simulink model "DATA_PERTURB_AND_OBSERVE_STEADY_STATE_IRRADIATION_VARIATION"  (R2023b)
settings: Solver=ode23  StartTime=0.0  StopTime=0.5  RelTol=1e-7
undefined symbols (not defined in the file): Acid, Lead
libraries: spsMeanLib x40, spsSeriesRLCBranchLib x25, spsVoltageMeasurementLib x20, spsCurrentMeasurementLib x10, spsBatteryLib x5, spsDiodeLib x5, spsMosfetLib x5, simulink x5, spsPVArrayLib x5, spsPWMGeneratorDCDCLib x5, sps_lib x1
settings Model: Creator=User  LastModifiedBy=D E L L
settings DebuggingCC: AlgebraicLoopMsg=none

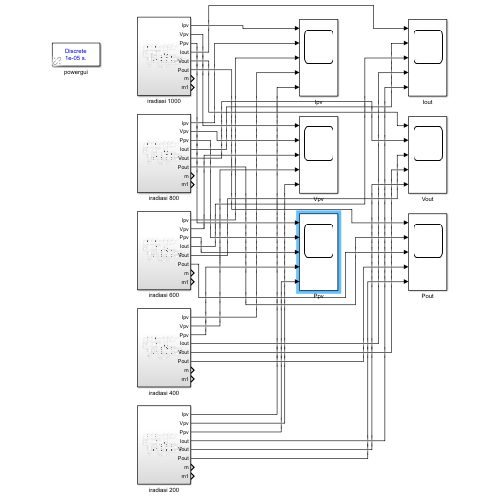
[thumbnail: Simulink's stored preview of the top-level diagram]
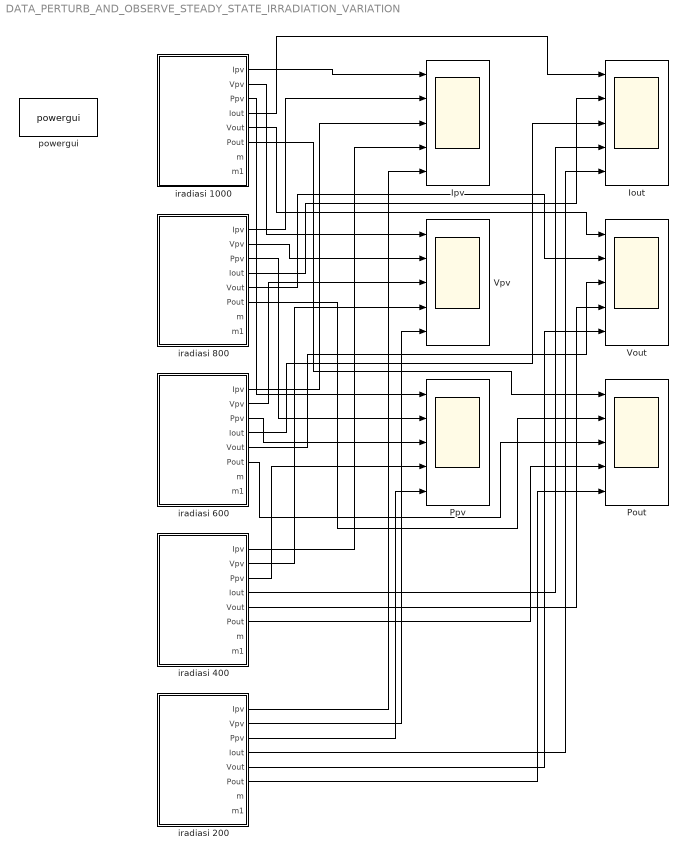
== system DATA_PERTURB_AND_OBSERVE_STEADY_STATE_IRRADIATION_VARIATION ==
  Iout : Scope  NumInputPorts=5
  Ipv : Scope  NumInputPorts=5
  Pout : Scope  NumInputPorts=5
  Ppv : Scope  NumInputPorts=5
  Vout : Scope  NumInputPorts=5
  Vpv : Scope  NumInputPorts=5
  iradiasi 1000 : Subsystem
  iradiasi 200 : Subsystem
  iradiasi 400 : Subsystem
  iradiasi 600 : Subsystem
  iradiasi 800 : Subsystem
  powergui : sps_lib/powergui  Priority=1  SimulationMode=Discrete  SampleTime=1e-05  frequency=60  Iterations=50  frequencyindice=0  Pbase=100e6  ErrMax=1e-4  UnitsV=kV  UnitsW=MW  buscounter=0  FunctionMessages=off  echomessages=off  EnableUseOfTLC=off  CurrentSourceSwitches=off  DisableSnubberDevices=off  DisableRonSwitches=off  DisableVfSwitches=off  DisplayEquations=off  AutomaticDiscreteSolvers=off  SolverType=Tustin/Backward Euler (TBE)  Interpol=off  ExternalGateDelay=off  methode=off  Ts=100  x0status=blocks  SPID=on  SwTol=0  HookPort=off  NonlinearTolerance=1e-4  nMaxIteration=100  ContinueOnMaxIteration=off  RestoreLinks=warning  ResistiveCurrentMeasurement=off  Frange=[0:2:500]  Ylog=off  Xlog=on  ShowGrid=off  save=off  variable=ZData  structure=0  ZoomFFT=off  StartTime=0.0  cycles=1  DisplayStyle=1  fundamental=60  FreqAxis=off  MaxFrequency=1000  frequencyindicesteady=1  RmsSteady=1  display=off
  wires:
  iradiasi 1000/1(Ipv) -> Ipv/1
  iradiasi 800/1(Ipv) -> Ipv/2
  iradiasi 600/1(Ipv) -> Ipv/3
  iradiasi 400/1(Ipv) -> Ipv/4
  iradiasi 200/1(Ipv) -> Ipv/5
  iradiasi 1000/2(Vpv) -> Vpv/1
  iradiasi 800/2(Vpv) -> Vpv/2
  iradiasi 600/2(Vpv) -> Vpv/3
  iradiasi 400/2(Vpv) -> Vpv/4
  iradiasi 200/2(Vpv) -> Vpv/5
  iradiasi 1000/3(Ppv) -> Ppv/1
  iradiasi 800/3(Ppv) -> Ppv/2
  iradiasi 600/3(Ppv) -> Ppv/3
  iradiasi 400/3(Ppv) -> Ppv/4
  iradiasi 200/3(Ppv) -> Ppv/5
  iradiasi 1000/4(Iout) -> Iout/1
  iradiasi 800/4(Iout) -> Iout/2
  iradiasi 600/4(Iout) -> Iout/3
  iradiasi 400/4(Iout) -> Iout/4
  iradiasi 200/4(Iout) -> Iout/5
  iradiasi 1000/5(Vout) -> Vout/1
  iradiasi 800/5(Vout) -> Vout/2
  iradiasi 600/5(Vout) -> Vout/3
  iradiasi 400/5(Vout) -> Vout/4
  iradiasi 200/5(Vout) -> Vout/5
  iradiasi 1000/6(Pout) -> Pout/1
  iradiasi 800/6(Pout) -> Pout/2
  iradiasi 600/6(Pout) -> Pout/3
  iradiasi 400/6(Pout) -> Pout/4
  iradiasi 200/6(Pout) -> Pout/5

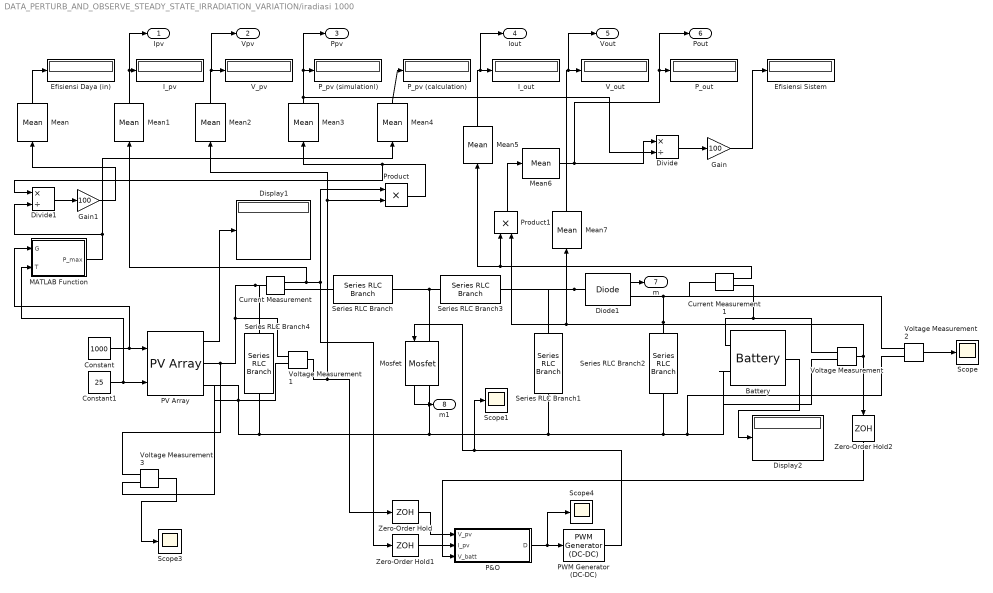
== system DATA_PERTURB_AND_OBSERVE_STEADY_STATE_IRRADIATION_VARIATION/iradiasi 1000 ==
  Battery : spsBatteryLib/Battery  BatType=Lead-Acid  ShowTempParam=off  ThermalPreset=no  ShowAgeParam=off  NomV=12  NomQ=3.5  SOC=90  Batt_Tr=1  PresetModel=off  MaxQ=3.125  MinV=9  FullV=14.4  Dis_rate=0.6  R=0.04  Normal_OP=0.93083  expZone="[12.2171         0.01]"  current=[6.5 13 32.5]  Units=Time  Tci=20  NomT=20  T2=-30  MaxQ2=4.8  FullV2=7.1  Normal_OP2=5.655  expZone2="[6.58           1]"  Rca=0.6  ti=2000  Dp=0  Neq0=0  Tsim=1e6  Ta1=25  Qeol=5.4*0.9  Reol=0.013333*1.2  Char_age=[2.3478, 3]  Dis_age=[2.3478, 10]  N1=1500  N2=10500  N3=1000  N4=1400  Ta2=45  N5=950
  Constant : Constant  Value=1000
  Constant1 : Constant  Value=25
  Current Measurement : spsCurrentMeasurementLib/Current Measurement  PhasorSimulation=off  OutputType=Complex  PSBequivalent=0
  Current Measurement1 : spsCurrentMeasurementLib/Current Measurement  PhasorSimulation=off  OutputType=Complex  PSBequivalent=0
  Diode1 : spsDiodeLib/Diode  Ron=0.001  Lon=0  Vf=0.4  IC=0  UseSnubber=0  Rs=500  Cs=250e-9  Measurements=on
  Display1 : Display
  Display2 : Display
  Divide : Product  Inputs=*/
  Divide1 : Product  Inputs=*/
  Efisiensi Daya (in) : Display
  Efisiensi Sistem : Display
  Gain : Gain  Gain=100
  Gain1 : Gain  Gain=100
  I_out : Display
  I_pv : Display
  MATLAB Function : MATLAB Function  TreatAsAtomicUnit=on
  Mean{,1..7} (8 alike) : spsMeanLib/Mean  Freq=60  Vinit=0  Ts=0
  Mosfet : spsMosfetLib/Mosfet  Ron=0.044  Lon=0  Rd=1.3  Vfd=0  IC=0  Rs=1e5  Cs=inf  Measurements=on
  P&O : Subsystem
  PV Array : spsPVArrayLib/PV Array  Npar=1  Nser=1  PlotType=array @ 1000 W/m2 & specified temperatures  S_vec="[ 1000  500  100 ]"  Temp_C_vec="[ 45 25  ]"  ModuleName=User-defined  PlotWhenSelected=off  Pm=10.08  Ncell=36  Voc=21.6  Isc=0.61  Vm=18  Im=0.56  beta_Voc_pc=-0.36099  alpha_Isc_pc=0.102  beta_Voc=-0.077974  alpha_Isc=0.0006222  IL=0.61115  I0=2.2544e-11  nI=0.97389  Rsh=828.4328  Rs=1.5603  RobustModel=off  RobustCellTemperature=313.3991  BAL=on  Tc=1e-6  Tfilter=1e-5
  PWM Generator (DC-DC) : spsPWMGeneratorDCDCLib/PWM Generator (DC-DC)  Fsw=31000  Ts=0
  P_out : Display
  P_pv (calculation) : Display
  P_pv (simulationl) : Display
  Product : Product
  Product1 : Product
  Scope{,1,3..4} (4 alike) : Scope
  Series RLC Branch : spsSeriesRLCBranchLib/Series RLC Branch  LConnTagsString=__new0  RConnTagsString=__new0  BranchType=L  Resistance=1  Inductance=1.5e-3  SetiL0=on  InitialCurrent=0.01  Capacitance=1e-6  Setx0=off  InitialVoltage=0  Measurements=None
  Series RLC Branch1 : spsSeriesRLCBranchLib/Series RLC Branch  LConnTagsString=__new0  RConnTagsString=__new0  BranchType=L  Resistance=1  Inductance=1.5e-3  SetiL0=on  InitialCurrent=0.01  Capacitance=1e-6  Setx0=off  InitialVoltage=0  Measurements=None
  Series RLC Branch2 : spsSeriesRLCBranchLib/Series RLC Branch  LConnTagsString=__new0  RConnTagsString=__new0  BranchType=C  Resistance=1  Inductance=1e-3  SetiL0=off  InitialCurrent=0  Capacitance=470e-6  Setx0=on  InitialVoltage=0.1  Measurements=None
  Series RLC Branch3 : spsSeriesRLCBranchLib/Series RLC Branch  LConnTagsString=__new0  RConnTagsString=__new0  BranchType=C  Resistance=1  Inductance=1e-3  SetiL0=off  InitialCurrent=0  Capacitance=22e-6  Setx0=off  InitialVoltage=0  Measurements=None
  Series RLC Branch4 : spsSeriesRLCBranchLib/Series RLC Branch  LConnTagsString=__new0  RConnTagsString=__new0  BranchType=C  Resistance=1  Inductance=1e-3  SetiL0=off  InitialCurrent=0  Capacitance=470e-6  Setx0=on  InitialVoltage=0.1  Measurements=None
  V_out : Display
  V_pv : Display
  Voltage Measurement{,1..3} (4 alike) : spsVoltageMeasurementLib/Voltage Measurement  PhasorSimulation=off  OutputType=Complex  PSBequivalent=0
  Zero-Order Hold : ZeroOrderHold  SampleTime=0.05
  Zero-Order Hold1 : ZeroOrderHold  SampleTime=0.05
  Zero-Order Hold2 : ZeroOrderHold  SampleTime=0.05
  Ipv : Outport
  Vpv : Outport  Port=2
  Ppv : Outport  Port=3
  Iout : Outport  Port=4
  Vout : Outport  Port=5
  Pout : Outport  Port=6
  m : Outport  Port=7
  m1 : Outport  Port=8
  wires:
  Mean1/1 -> Ipv/1, I_pv/1
  Mean2/1 -> Vpv/1, V_pv/1
  PWM Generator (DC-DC)/1 -> Scope1/1, Mosfet/1
  Divide/1 -> Gain/1
  Current Measurement1/1 -> Product1/1, Mean5/1
  Constant1/1 -> MATLAB Function/2(T), PV Array/2
  Constant/1 -> MATLAB Function/1(G), PV Array/1
  Divide1/1 -> Gain1/1
  Gain1/1 -> Mean/1
  Voltage Measurement2/1 -> Scope/1
  Voltage Measurement/1 -> Product1/2, Mean7/1, Zero-Order Hold2/1
  Diode1/1 -> m/1
  Gain/1 -> Efisiensi Sistem/1
  P&O/1(D) -> Scope4/1, PWM Generator (DC-DC)/1
  Product/1 -> Mean3/1, Divide1/1
  Voltage Measurement1/1 -> Zero-Order Hold/1, Mean2/1, Product/2
  Current Measurement/1 -> Zero-Order Hold1/1, Product/1, Mean1/1
  Mean6/1 -> Divide/1, Pout/1, P_out/1
  Mean4/1 -> P_pv (calculation)/1
  Zero-Order Hold2/1 -> P&O/3(V_batt)
  Product1/1 -> Mean6/1
  Zero-Order Hold1/1 -> P&O/2(I_pv)
  Mean3/1 -> Ppv/1, P_pv (simulationl)/1, Divide/2
  Zero-Order Hold/1 -> P&O/1(V_pv)
  Mean5/1 -> Iout/1, I_out/1
  Voltage Measurement3/1 -> Scope3/1
  Mean7/1 -> Vout/1, V_out/1
  MATLAB Function/1(P_max) -> Mean4/1, Divide1/2
  Battery/1 -> Display2/1
  PV Array/1 -> Display1/1
  Mean/1 -> Efisiensi Daya (in)/1
  Mosfet/1 -> m1/1
  connections:
  Diode1/LConn1 -- Series RLC Branch3/RConn1 -- Series RLC Branch1/LConn1
  Series RLC Branch1/RConn1 -- Series RLC Branch4/RConn1 -- Voltage Measurement3/LConn2 -- PV Array/RConn2 -- Voltage Measurement1/LConn2 -- Mosfet/RConn1 -- Voltage Measurement2/LConn2 -- Voltage Measurement/LConn2 -- Battery/LConn2 -- Series RLC Branch2/RConn1
  PV Array/RConn1 -- Voltage Measurement3/LConn1 -- Voltage Measurement1/LConn1 -- Series RLC Branch4/LConn1 -- Current Measurement/LConn1
  Series RLC Branch3/LConn1 -- Series RLC Branch/RConn1 -- Mosfet/LConn1
  Series RLC Branch2/LConn1 -- Current Measurement1/LConn1 -- Voltage Measurement2/LConn1 -- Diode1/RConn1
  Current Measurement/RConn1 -- Series RLC Branch/LConn1
  Current Measurement1/RConn1 -- Voltage Measurement/LConn1 -- Battery/LConn1

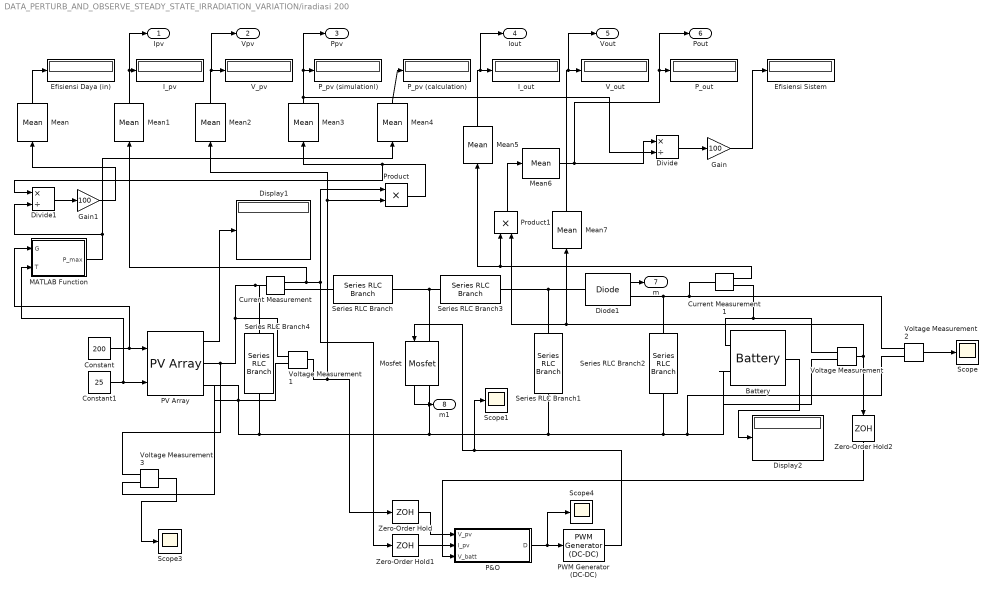
== system DATA_PERTURB_AND_OBSERVE_STEADY_STATE_IRRADIATION_VARIATION/iradiasi 200 ==
  Battery : spsBatteryLib/Battery  BatType=Lead-Acid  ShowTempParam=off  ThermalPreset=no  ShowAgeParam=off  NomV=12  NomQ=3.5  SOC=90  Batt_Tr=1  PresetModel=off  MaxQ=3.125  MinV=9  FullV=14.4  Dis_rate=0.6  R=0.04  Normal_OP=0.93083  expZone="[12.2171         0.01]"  current=[6.5 13 32.5]  Units=Time  Tci=20  NomT=20  T2=-30  MaxQ2=4.8  FullV2=7.1  Normal_OP2=5.655  expZone2="[6.58           1]"  Rca=0.6  ti=2000  Dp=0  Neq0=0  Tsim=1e6  Ta1=25  Qeol=5.4*0.9  Reol=0.013333*1.2  Char_age=[2.3478, 3]  Dis_age=[2.3478, 10]  N1=1500  N2=10500  N3=1000  N4=1400  Ta2=45  N5=950
  Constant : Constant  Value=200
  Constant1 : Constant  Value=25
  Current Measurement : spsCurrentMeasurementLib/Current Measurement  PhasorSimulation=off  OutputType=Complex  PSBequivalent=0
  Current Measurement1 : spsCurrentMeasurementLib/Current Measurement  PhasorSimulation=off  OutputType=Complex  PSBequivalent=0
  Diode1 : spsDiodeLib/Diode  Ron=0.001  Lon=0  Vf=0.4  IC=0  UseSnubber=0  Rs=500  Cs=250e-9  Measurements=on
  Display1 : Display
  Display2 : Display
  Divide : Product  Inputs=*/
  Divide1 : Product  Inputs=*/
  Efisiensi Daya (in) : Display
  Efisiensi Sistem : Display
  Gain : Gain  Gain=100
  Gain1 : Gain  Gain=100
  I_out : Display
  I_pv : Display
  MATLAB Function : MATLAB Function  TreatAsAtomicUnit=on
  Mean{,1..7} (8 alike) : spsMeanLib/Mean  Freq=60  Vinit=0  Ts=0
  Mosfet : spsMosfetLib/Mosfet  Ron=0.044  Lon=0  Rd=1.3  Vfd=0  IC=0  Rs=1e5  Cs=inf  Measurements=on
  P&O : Subsystem
  PV Array : spsPVArrayLib/PV Array  Npar=1  Nser=1  PlotType=array @ 1000 W/m2 & specified temperatures  S_vec="[ 1000  500  100 ]"  Temp_C_vec="[ 45 25  ]"  ModuleName=User-defined  PlotWhenSelected=off  Pm=10.08  Ncell=36  Voc=21.6  Isc=0.61  Vm=18  Im=0.56  beta_Voc_pc=-0.36099  alpha_Isc_pc=0.102  beta_Voc=-0.077974  alpha_Isc=0.0006222  IL=0.61115  I0=2.2544e-11  nI=0.97389  Rsh=828.4328  Rs=1.5603  RobustModel=off  RobustCellTemperature=313.3991  BAL=on  Tc=1e-6  Tfilter=1e-5
  PWM Generator (DC-DC) : spsPWMGeneratorDCDCLib/PWM Generator (DC-DC)  Fsw=31000  Ts=0
  P_out : Display
  P_pv (calculation) : Display
  P_pv (simulationl) : Display
  Product : Product
  Product1 : Product
  Scope{,1,3..4} (4 alike) : Scope
  Series RLC Branch : spsSeriesRLCBranchLib/Series RLC Branch  LConnTagsString=__new0  RConnTagsString=__new0  BranchType=L  Resistance=1  Inductance=1.5e-3  SetiL0=on  InitialCurrent=0.01  Capacitance=1e-6  Setx0=off  InitialVoltage=0  Measurements=None
  Series RLC Branch1 : spsSeriesRLCBranchLib/Series RLC Branch  LConnTagsString=__new0  RConnTagsString=__new0  BranchType=L  Resistance=1  Inductance=1.5e-3  SetiL0=on  InitialCurrent=0.01  Capacitance=1e-6  Setx0=off  InitialVoltage=0  Measurements=None
  Series RLC Branch2 : spsSeriesRLCBranchLib/Series RLC Branch  LConnTagsString=__new0  RConnTagsString=__new0  BranchType=C  Resistance=1  Inductance=1e-3  SetiL0=off  InitialCurrent=0  Capacitance=470e-6  Setx0=on  InitialVoltage=0.1  Measurements=None
  Series RLC Branch3 : spsSeriesRLCBranchLib/Series RLC Branch  LConnTagsString=__new0  RConnTagsString=__new0  BranchType=C  Resistance=1  Inductance=1e-3  SetiL0=off  InitialCurrent=0  Capacitance=22e-6  Setx0=off  InitialVoltage=0  Measurements=None
  Series RLC Branch4 : spsSeriesRLCBranchLib/Series RLC Branch  LConnTagsString=__new0  RConnTagsString=__new0  BranchType=C  Resistance=1  Inductance=1e-3  SetiL0=off  InitialCurrent=0  Capacitance=470e-6  Setx0=on  InitialVoltage=0.1  Measurements=None
  V_out : Display
  V_pv : Display
  Voltage Measurement{,1..3} (4 alike) : spsVoltageMeasurementLib/Voltage Measurement  PhasorSimulation=off  OutputType=Complex  PSBequivalent=0
  Zero-Order Hold : ZeroOrderHold  SampleTime=0.05
  Zero-Order Hold1 : ZeroOrderHold  SampleTime=0.05
  Zero-Order Hold2 : ZeroOrderHold  SampleTime=0.05
  Ipv : Outport
  Vpv : Outport  Port=2
  Ppv : Outport  Port=3
  Iout : Outport  Port=4
  Vout : Outport  Port=5
  Pout : Outport  Port=6
  m : Outport  Port=7
  m1 : Outport  Port=8
  wires:
  Mean1/1 -> Ipv/1, I_pv/1
  Mean2/1 -> Vpv/1, V_pv/1
  PWM Generator (DC-DC)/1 -> Scope1/1, Mosfet/1
  Divide/1 -> Gain/1
  Current Measurement1/1 -> Product1/1, Mean5/1
  Constant1/1 -> MATLAB Function/2(T), PV Array/2
  Constant/1 -> MATLAB Function/1(G), PV Array/1
  Divide1/1 -> Gain1/1
  Gain1/1 -> Mean/1
  Voltage Measurement2/1 -> Scope/1
  Voltage Measurement/1 -> Product1/2, Mean7/1, Zero-Order Hold2/1
  Diode1/1 -> m/1
  Gain/1 -> Efisiensi Sistem/1
  P&O/1(D) -> Scope4/1, PWM Generator (DC-DC)/1
  Product/1 -> Mean3/1, Divide1/1
  Voltage Measurement1/1 -> Zero-Order Hold/1, Mean2/1, Product/2
  Current Measurement/1 -> Zero-Order Hold1/1, Product/1, Mean1/1
  Mean6/1 -> Divide/1, Pout/1, P_out/1
  Mean4/1 -> P_pv (calculation)/1
  Zero-Order Hold2/1 -> P&O/3(V_batt)
  Product1/1 -> Mean6/1
  Zero-Order Hold1/1 -> P&O/2(I_pv)
  Mean3/1 -> Ppv/1, P_pv (simulationl)/1, Divide/2
  Zero-Order Hold/1 -> P&O/1(V_pv)
  Mean5/1 -> Iout/1, I_out/1
  Voltage Measurement3/1 -> Scope3/1
  Mean7/1 -> Vout/1, V_out/1
  MATLAB Function/1(P_max) -> Mean4/1, Divide1/2
  Battery/1 -> Display2/1
  PV Array/1 -> Display1/1
  Mean/1 -> Efisiensi Daya (in)/1
  Mosfet/1 -> m1/1
  connections:
  Series RLC Branch3/RConn1 -- Diode1/LConn1 -- Series RLC Branch1/LConn1
  Series RLC Branch1/RConn1 -- Series RLC Branch4/RConn1 -- Voltage Measurement3/LConn2 -- PV Array/RConn2 -- Voltage Measurement1/LConn2 -- Mosfet/RConn1 -- Voltage Measurement2/LConn2 -- Voltage Measurement/LConn2 -- Battery/LConn2 -- Series RLC Branch2/RConn1
  PV Array/RConn1 -- Voltage Measurement3/LConn1 -- Voltage Measurement1/LConn1 -- Series RLC Branch4/LConn1 -- Current Measurement/LConn1
  Series RLC Branch/RConn1 -- Series RLC Branch3/LConn1 -- Mosfet/LConn1
  Current Measurement1/LConn1 -- Voltage Measurement2/LConn1 -- Series RLC Branch2/LConn1 -- Diode1/RConn1
  Current Measurement/RConn1 -- Series RLC Branch/LConn1
  Current Measurement1/RConn1 -- Voltage Measurement/LConn1 -- Battery/LConn1

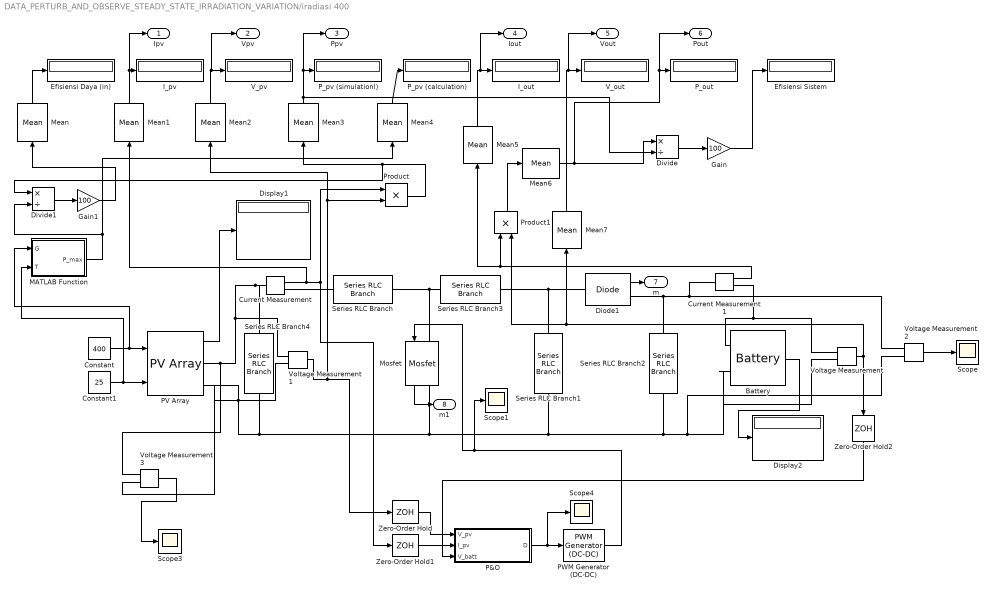
== system DATA_PERTURB_AND_OBSERVE_STEADY_STATE_IRRADIATION_VARIATION/iradiasi 400 ==
  Battery : spsBatteryLib/Battery  BatType=Lead-Acid  ShowTempParam=off  ThermalPreset=no  ShowAgeParam=off  NomV=12  NomQ=3.5  SOC=90  Batt_Tr=1  PresetModel=off  MaxQ=3.125  MinV=9  FullV=14.4  Dis_rate=0.6  R=0.04  Normal_OP=0.93083  expZone="[12.2171         0.01]"  current=[6.5 13 32.5]  Units=Time  Tci=20  NomT=20  T2=-30  MaxQ2=4.8  FullV2=7.1  Normal_OP2=5.655  expZone2="[6.58           1]"  Rca=0.6  ti=2000  Dp=0  Neq0=0  Tsim=1e6  Ta1=25  Qeol=5.4*0.9  Reol=0.013333*1.2  Char_age=[2.3478, 3]  Dis_age=[2.3478, 10]  N1=1500  N2=10500  N3=1000  N4=1400  Ta2=45  N5=950
  Constant : Constant  Value=400
  Constant1 : Constant  Value=25
  Current Measurement : spsCurrentMeasurementLib/Current Measurement  PhasorSimulation=off  OutputType=Complex  PSBequivalent=0
  Current Measurement1 : spsCurrentMeasurementLib/Current Measurement  PhasorSimulation=off  OutputType=Complex  PSBequivalent=0
  Diode1 : spsDiodeLib/Diode  Ron=0.001  Lon=0  Vf=0.4  IC=0  UseSnubber=0  Rs=500  Cs=250e-9  Measurements=on
  Display1 : Display
  Display2 : Display
  Divide : Product  Inputs=*/
  Divide1 : Product  Inputs=*/
  Efisiensi Daya (in) : Display
  Efisiensi Sistem : Display
  Gain : Gain  Gain=100
  Gain1 : Gain  Gain=100
  I_out : Display
  I_pv : Display
  MATLAB Function : MATLAB Function  TreatAsAtomicUnit=on
  Mean{,1..7} (8 alike) : spsMeanLib/Mean  Freq=60  Vinit=0  Ts=0
  Mosfet : spsMosfetLib/Mosfet  Ron=0.044  Lon=0  Rd=1.3  Vfd=0  IC=0  Rs=1e5  Cs=inf  Measurements=on
  P&O : Subsystem
  PV Array : spsPVArrayLib/PV Array  Npar=1  Nser=1  PlotType=array @ 1000 W/m2 & specified temperatures  S_vec="[ 1000  500  100 ]"  Temp_C_vec="[ 45 25  ]"  ModuleName=User-defined  PlotWhenSelected=off  Pm=10.08  Ncell=36  Voc=21.6  Isc=0.61  Vm=18  Im=0.56  beta_Voc_pc=-0.36099  alpha_Isc_pc=0.102  beta_Voc=-0.077974  alpha_Isc=0.0006222  IL=0.61115  I0=2.2544e-11  nI=0.97389  Rsh=828.4328  Rs=1.5603  RobustModel=off  RobustCellTemperature=313.3991  BAL=on  Tc=1e-6  Tfilter=1e-5
  PWM Generator (DC-DC) : spsPWMGeneratorDCDCLib/PWM Generator (DC-DC)  Fsw=31000  Ts=0
  P_out : Display
  P_pv (calculation) : Display
  P_pv (simulationl) : Display
  Product : Product
  Product1 : Product
  Scope{,1,3..4} (4 alike) : Scope
  Series RLC Branch : spsSeriesRLCBranchLib/Series RLC Branch  LConnTagsString=__new0  RConnTagsString=__new0  BranchType=L  Resistance=1  Inductance=1.5e-3  SetiL0=on  InitialCurrent=0.01  Capacitance=1e-6  Setx0=off  InitialVoltage=0  Measurements=None
  Series RLC Branch1 : spsSeriesRLCBranchLib/Series RLC Branch  LConnTagsString=__new0  RConnTagsString=__new0  BranchType=L  Resistance=1  Inductance=1.5e-3  SetiL0=on  InitialCurrent=0.01  Capacitance=1e-6  Setx0=off  InitialVoltage=0  Measurements=None
  Series RLC Branch2 : spsSeriesRLCBranchLib/Series RLC Branch  LConnTagsString=__new0  RConnTagsString=__new0  BranchType=C  Resistance=1  Inductance=1e-3  SetiL0=off  InitialCurrent=0  Capacitance=470e-6  Setx0=on  InitialVoltage=0.1  Measurements=None
  Series RLC Branch3 : spsSeriesRLCBranchLib/Series RLC Branch  LConnTagsString=__new0  RConnTagsString=__new0  BranchType=C  Resistance=1  Inductance=1e-3  SetiL0=off  InitialCurrent=0  Capacitance=22e-6  Setx0=off  InitialVoltage=0  Measurements=None
  Series RLC Branch4 : spsSeriesRLCBranchLib/Series RLC Branch  LConnTagsString=__new0  RConnTagsString=__new0  BranchType=C  Resistance=1  Inductance=1e-3  SetiL0=off  InitialCurrent=0  Capacitance=470e-6  Setx0=on  InitialVoltage=0.1  Measurements=None
  V_out : Display
  V_pv : Display
  Voltage Measurement{,1..3} (4 alike) : spsVoltageMeasurementLib/Voltage Measurement  PhasorSimulation=off  OutputType=Complex  PSBequivalent=0
  Zero-Order Hold : ZeroOrderHold  SampleTime=0.05
  Zero-Order Hold1 : ZeroOrderHold  SampleTime=0.05
  Zero-Order Hold2 : ZeroOrderHold  SampleTime=0.05
  Ipv : Outport
  Vpv : Outport  Port=2
  Ppv : Outport  Port=3
  Iout : Outport  Port=4
  Vout : Outport  Port=5
  Pout : Outport  Port=6
  m : Outport  Port=7
  m1 : Outport  Port=8
  wires:
  Mean1/1 -> Ipv/1, I_pv/1
  Mean2/1 -> Vpv/1, V_pv/1
  PWM Generator (DC-DC)/1 -> Scope1/1, Mosfet/1
  Divide/1 -> Gain/1
  Current Measurement1/1 -> Product1/1, Mean5/1
  Constant1/1 -> MATLAB Function/2(T), PV Array/2
  Constant/1 -> MATLAB Function/1(G), PV Array/1
  Divide1/1 -> Gain1/1
  Gain1/1 -> Mean/1
  Voltage Measurement2/1 -> Scope/1
  Voltage Measurement/1 -> Product1/2, Mean7/1, Zero-Order Hold2/1
  Diode1/1 -> m/1
  Gain/1 -> Efisiensi Sistem/1
  P&O/1(D) -> Scope4/1, PWM Generator (DC-DC)/1
  Product/1 -> Mean3/1, Divide1/1
  Voltage Measurement1/1 -> Zero-Order Hold/1, Mean2/1, Product/2
  Current Measurement/1 -> Zero-Order Hold1/1, Product/1, Mean1/1
  Mean6/1 -> Divide/1, Pout/1, P_out/1
  Mean4/1 -> P_pv (calculation)/1
  Zero-Order Hold2/1 -> P&O/3(V_batt)
  Product1/1 -> Mean6/1
  Zero-Order Hold1/1 -> P&O/2(I_pv)
  Mean3/1 -> Ppv/1, P_pv (simulationl)/1, Divide/2
  Zero-Order Hold/1 -> P&O/1(V_pv)
  Mean5/1 -> Iout/1, I_out/1
  Voltage Measurement3/1 -> Scope3/1
  Mean7/1 -> Vout/1, V_out/1
  MATLAB Function/1(P_max) -> Mean4/1, Divide1/2
  Battery/1 -> Display2/1
  PV Array/1 -> Display1/1
  Mean/1 -> Efisiensi Daya (in)/1
  Mosfet/1 -> m1/1
  connections:
  Series RLC Branch3/RConn1 -- Diode1/LConn1 -- Series RLC Branch1/LConn1
  Series RLC Branch1/RConn1 -- Series RLC Branch4/RConn1 -- Voltage Measurement3/LConn2 -- PV Array/RConn2 -- Voltage Measurement1/LConn2 -- Mosfet/RConn1 -- Voltage Measurement2/LConn2 -- Voltage Measurement/LConn2 -- Battery/LConn2 -- Series RLC Branch2/RConn1
  PV Array/RConn1 -- Voltage Measurement3/LConn1 -- Voltage Measurement1/LConn1 -- Series RLC Branch4/LConn1 -- Current Measurement/LConn1
  Series RLC Branch/RConn1 -- Series RLC Branch3/LConn1 -- Mosfet/LConn1
  Current Measurement1/LConn1 -- Voltage Measurement2/LConn1 -- Series RLC Branch2/LConn1 -- Diode1/RConn1
  Current Measurement/RConn1 -- Series RLC Branch/LConn1
  Current Measurement1/RConn1 -- Voltage Measurement/LConn1 -- Battery/LConn1

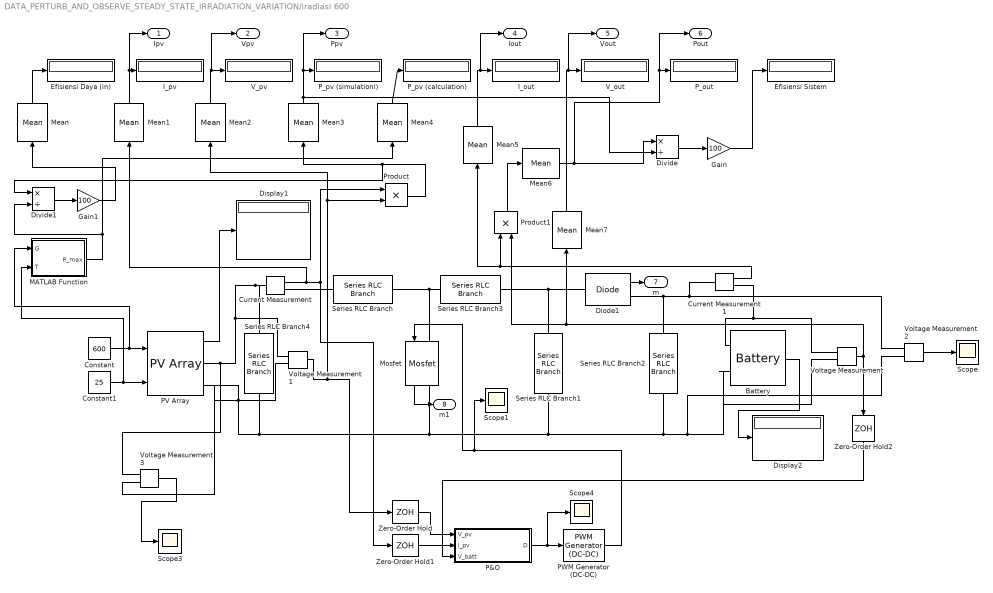
== system DATA_PERTURB_AND_OBSERVE_STEADY_STATE_IRRADIATION_VARIATION/iradiasi 600 ==
  Battery : spsBatteryLib/Battery  BatType=Lead-Acid  ShowTempParam=off  ThermalPreset=no  ShowAgeParam=off  NomV=12  NomQ=3.5  SOC=90  Batt_Tr=1  PresetModel=off  MaxQ=3.125  MinV=9  FullV=14.4  Dis_rate=0.6  R=0.04  Normal_OP=0.93083  expZone="[12.2171         0.01]"  current=[6.5 13 32.5]  Units=Time  Tci=20  NomT=20  T2=-30  MaxQ2=4.8  FullV2=7.1  Normal_OP2=5.655  expZone2="[6.58           1]"  Rca=0.6  ti=2000  Dp=0  Neq0=0  Tsim=1e6  Ta1=25  Qeol=5.4*0.9  Reol=0.013333*1.2  Char_age=[2.3478, 3]  Dis_age=[2.3478, 10]  N1=1500  N2=10500  N3=1000  N4=1400  Ta2=45  N5=950
  Constant : Constant  Value=600
  Constant1 : Constant  Value=25
  Current Measurement : spsCurrentMeasurementLib/Current Measurement  PhasorSimulation=off  OutputType=Complex  PSBequivalent=0
  Current Measurement1 : spsCurrentMeasurementLib/Current Measurement  PhasorSimulation=off  OutputType=Complex  PSBequivalent=0
  Diode1 : spsDiodeLib/Diode  Ron=0.001  Lon=0  Vf=0.4  IC=0  UseSnubber=0  Rs=500  Cs=250e-9  Measurements=on
  Display1 : Display
  Display2 : Display
  Divide : Product  Inputs=*/
  Divide1 : Product  Inputs=*/
  Efisiensi Daya (in) : Display
  Efisiensi Sistem : Display
  Gain : Gain  Gain=100
  Gain1 : Gain  Gain=100
  I_out : Display
  I_pv : Display
  MATLAB Function : MATLAB Function  TreatAsAtomicUnit=on
  Mean{,1..7} (8 alike) : spsMeanLib/Mean  Freq=60  Vinit=0  Ts=0
  Mosfet : spsMosfetLib/Mosfet  Ron=0.044  Lon=0  Rd=1.3  Vfd=0  IC=0  Rs=1e5  Cs=inf  Measurements=on
  P&O : Subsystem
  PV Array : spsPVArrayLib/PV Array  Npar=1  Nser=1  PlotType=array @ 1000 W/m2 & specified temperatures  S_vec="[ 1000  500  100 ]"  Temp_C_vec="[ 45 25  ]"  ModuleName=User-defined  PlotWhenSelected=off  Pm=10.08  Ncell=36  Voc=21.6  Isc=0.61  Vm=18  Im=0.56  beta_Voc_pc=-0.36099  alpha_Isc_pc=0.102  beta_Voc=-0.077974  alpha_Isc=0.0006222  IL=0.61115  I0=2.2544e-11  nI=0.97389  Rsh=828.4328  Rs=1.5603  RobustModel=off  RobustCellTemperature=313.3991  BAL=on  Tc=1e-6  Tfilter=1e-5
  PWM Generator (DC-DC) : spsPWMGeneratorDCDCLib/PWM Generator (DC-DC)  Fsw=31000  Ts=0
  P_out : Display
  P_pv (calculation) : Display
  P_pv (simulationl) : Display
  Product : Product
  Product1 : Product
  Scope{,1,3..4} (4 alike) : Scope
  Series RLC Branch : spsSeriesRLCBranchLib/Series RLC Branch  LConnTagsString=__new0  RConnTagsString=__new0  BranchType=L  Resistance=1  Inductance=1.5e-3  SetiL0=on  InitialCurrent=0.01  Capacitance=1e-6  Setx0=off  InitialVoltage=0  Measurements=None
  Series RLC Branch1 : spsSeriesRLCBranchLib/Series RLC Branch  LConnTagsString=__new0  RConnTagsString=__new0  BranchType=L  Resistance=1  Inductance=1.5e-3  SetiL0=on  InitialCurrent=0.01  Capacitance=1e-6  Setx0=off  InitialVoltage=0  Measurements=None
  Series RLC Branch2 : spsSeriesRLCBranchLib/Series RLC Branch  LConnTagsString=__new0  RConnTagsString=__new0  BranchType=C  Resistance=1  Inductance=1e-3  SetiL0=off  InitialCurrent=0  Capacitance=470e-6  Setx0=on  InitialVoltage=0.1  Measurements=None
  Series RLC Branch3 : spsSeriesRLCBranchLib/Series RLC Branch  LConnTagsString=__new0  RConnTagsString=__new0  BranchType=C  Resistance=1  Inductance=1e-3  SetiL0=off  InitialCurrent=0  Capacitance=22e-6  Setx0=off  InitialVoltage=0  Measurements=None
  Series RLC Branch4 : spsSeriesRLCBranchLib/Series RLC Branch  LConnTagsString=__new0  RConnTagsString=__new0  BranchType=C  Resistance=1  Inductance=1e-3  SetiL0=off  InitialCurrent=0  Capacitance=470e-6  Setx0=on  InitialVoltage=0.1  Measurements=None
  V_out : Display
  V_pv : Display
  Voltage Measurement{,1..3} (4 alike) : spsVoltageMeasurementLib/Voltage Measurement  PhasorSimulation=off  OutputType=Complex  PSBequivalent=0
  Zero-Order Hold : ZeroOrderHold  SampleTime=0.05
  Zero-Order Hold1 : ZeroOrderHold  SampleTime=0.05
  Zero-Order Hold2 : ZeroOrderHold  SampleTime=0.05
  Ipv : Outport
  Vpv : Outport  Port=2
  Ppv : Outport  Port=3
  Iout : Outport  Port=4
  Vout : Outport  Port=5
  Pout : Outport  Port=6
  m : Outport  Port=7
  m1 : Outport  Port=8
  wires:
  Mean1/1 -> Ipv/1, I_pv/1
  Mean2/1 -> Vpv/1, V_pv/1
  PWM Generator (DC-DC)/1 -> Scope1/1, Mosfet/1
  Divide/1 -> Gain/1
  Current Measurement1/1 -> Product1/1, Mean5/1
  Constant1/1 -> MATLAB Function/2(T), PV Array/2
  Constant/1 -> MATLAB Function/1(G), PV Array/1
  Divide1/1 -> Gain1/1
  Gain1/1 -> Mean/1
  Voltage Measurement2/1 -> Scope/1
  Voltage Measurement/1 -> Product1/2, Mean7/1, Zero-Order Hold2/1
  Diode1/1 -> m/1
  Gain/1 -> Efisiensi Sistem/1
  P&O/1(D) -> Scope4/1, PWM Generator (DC-DC)/1
  Product/1 -> Mean3/1, Divide1/1
  Voltage Measurement1/1 -> Zero-Order Hold/1, Mean2/1, Product/2
  Current Measurement/1 -> Zero-Order Hold1/1, Product/1, Mean1/1
  Mean6/1 -> Divide/1, Pout/1, P_out/1
  Mean4/1 -> P_pv (calculation)/1
  Zero-Order Hold2/1 -> P&O/3(V_batt)
  Product1/1 -> Mean6/1
  Zero-Order Hold1/1 -> P&O/2(I_pv)
  Mean3/1 -> Ppv/1, P_pv (simulationl)/1, Divide/2
  Zero-Order Hold/1 -> P&O/1(V_pv)
  Mean5/1 -> Iout/1, I_out/1
  Voltage Measurement3/1 -> Scope3/1
  Mean7/1 -> Vout/1, V_out/1
  MATLAB Function/1(P_max) -> Mean4/1, Divide1/2
  Battery/1 -> Display2/1
  PV Array/1 -> Display1/1
  Mean/1 -> Efisiensi Daya (in)/1
  Mosfet/1 -> m1/1
  connections:
  Series RLC Branch3/RConn1 -- Diode1/LConn1 -- Series RLC Branch1/LConn1
  Series RLC Branch1/RConn1 -- Series RLC Branch4/RConn1 -- Voltage Measurement3/LConn2 -- PV Array/RConn2 -- Voltage Measurement1/LConn2 -- Mosfet/RConn1 -- Voltage Measurement2/LConn2 -- Voltage Measurement/LConn2 -- Battery/LConn2 -- Series RLC Branch2/RConn1
  PV Array/RConn1 -- Voltage Measurement3/LConn1 -- Voltage Measurement1/LConn1 -- Series RLC Branch4/LConn1 -- Current Measurement/LConn1
  Series RLC Branch/RConn1 -- Series RLC Branch3/LConn1 -- Mosfet/LConn1
  Current Measurement1/LConn1 -- Voltage Measurement2/LConn1 -- Series RLC Branch2/LConn1 -- Diode1/RConn1
  Current Measurement/RConn1 -- Series RLC Branch/LConn1
  Current Measurement1/RConn1 -- Voltage Measurement/LConn1 -- Battery/LConn1

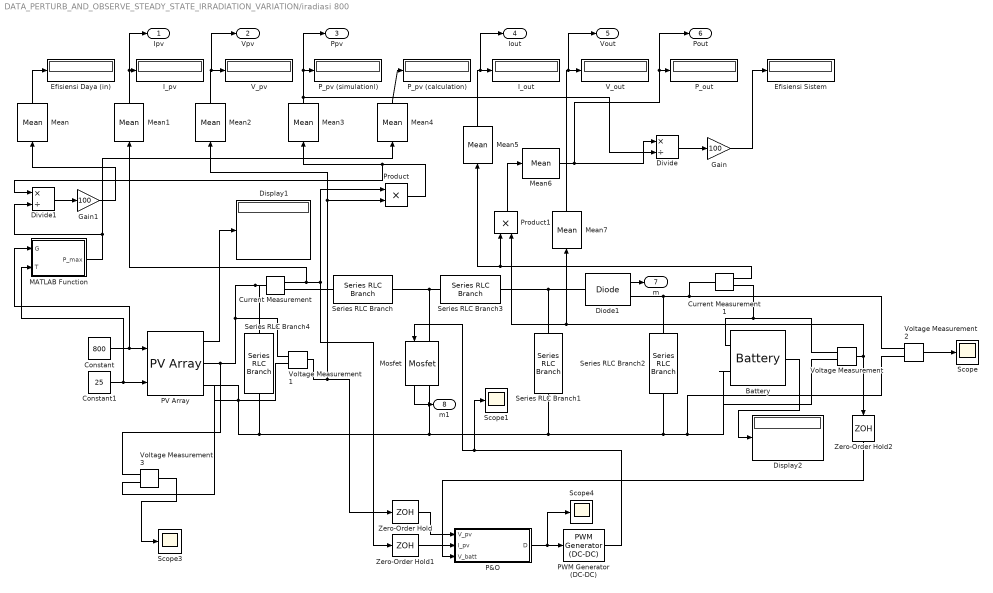
== system DATA_PERTURB_AND_OBSERVE_STEADY_STATE_IRRADIATION_VARIATION/iradiasi 800 ==
  Battery : spsBatteryLib/Battery  BatType=Lead-Acid  ShowTempParam=off  ThermalPreset=no  ShowAgeParam=off  NomV=12  NomQ=3.5  SOC=90  Batt_Tr=1  PresetModel=off  MaxQ=3.125  MinV=9  FullV=14.4  Dis_rate=0.6  R=0.04  Normal_OP=0.93083  expZone="[12.2171         0.01]"  current=[6.5 13 32.5]  Units=Time  Tci=20  NomT=20  T2=-30  MaxQ2=4.8  FullV2=7.1  Normal_OP2=5.655  expZone2="[6.58           1]"  Rca=0.6  ti=2000  Dp=0  Neq0=0  Tsim=1e6  Ta1=25  Qeol=5.4*0.9  Reol=0.013333*1.2  Char_age=[2.3478, 3]  Dis_age=[2.3478, 10]  N1=1500  N2=10500  N3=1000  N4=1400  Ta2=45  N5=950
  Constant : Constant  Value=800
  Constant1 : Constant  Value=25
  Current Measurement : spsCurrentMeasurementLib/Current Measurement  PhasorSimulation=off  OutputType=Complex  PSBequivalent=0
  Current Measurement1 : spsCurrentMeasurementLib/Current Measurement  PhasorSimulation=off  OutputType=Complex  PSBequivalent=0
  Diode1 : spsDiodeLib/Diode  Ron=0.001  Lon=0  Vf=0.4  IC=0  UseSnubber=0  Rs=500  Cs=250e-9  Measurements=on
  Display1 : Display
  Display2 : Display
  Divide : Product  Inputs=*/
  Divide1 : Product  Inputs=*/
  Efisiensi Daya (in) : Display
  Efisiensi Sistem : Display
  Gain : Gain  Gain=100
  Gain1 : Gain  Gain=100
  I_out : Display
  I_pv : Display
  MATLAB Function : MATLAB Function  TreatAsAtomicUnit=on
  Mean{,1..7} (8 alike) : spsMeanLib/Mean  Freq=60  Vinit=0  Ts=0
  Mosfet : spsMosfetLib/Mosfet  Ron=0.044  Lon=0  Rd=1.3  Vfd=0  IC=0  Rs=1e5  Cs=inf  Measurements=on
  P&O : Subsystem
  PV Array : spsPVArrayLib/PV Array  Npar=1  Nser=1  PlotType=array @ 1000 W/m2 & specified temperatures  S_vec="[ 1000  500  100 ]"  Temp_C_vec="[ 45 25  ]"  ModuleName=User-defined  PlotWhenSelected=off  Pm=10.08  Ncell=36  Voc=21.6  Isc=0.61  Vm=18  Im=0.56  beta_Voc_pc=-0.36099  alpha_Isc_pc=0.102  beta_Voc=-0.077974  alpha_Isc=0.0006222  IL=0.61115  I0=2.2544e-11  nI=0.97389  Rsh=828.4328  Rs=1.5603  RobustModel=off  RobustCellTemperature=313.3991  BAL=on  Tc=1e-6  Tfilter=1e-5
  PWM Generator (DC-DC) : spsPWMGeneratorDCDCLib/PWM Generator (DC-DC)  Fsw=31000  Ts=0
  P_out : Display
  P_pv (calculation) : Display
  P_pv (simulationl) : Display
  Product : Product
  Product1 : Product
  Scope{,1,3..4} (4 alike) : Scope
  Series RLC Branch : spsSeriesRLCBranchLib/Series RLC Branch  LConnTagsString=__new0  RConnTagsString=__new0  BranchType=L  Resistance=1  Inductance=1.5e-3  SetiL0=on  InitialCurrent=0.01  Capacitance=1e-6  Setx0=off  InitialVoltage=0  Measurements=None
  Series RLC Branch1 : spsSeriesRLCBranchLib/Series RLC Branch  LConnTagsString=__new0  RConnTagsString=__new0  BranchType=L  Resistance=1  Inductance=1.5e-3  SetiL0=on  InitialCurrent=0.01  Capacitance=1e-6  Setx0=off  InitialVoltage=0  Measurements=None
  Series RLC Branch2 : spsSeriesRLCBranchLib/Series RLC Branch  LConnTagsString=__new0  RConnTagsString=__new0  BranchType=C  Resistance=1  Inductance=1e-3  SetiL0=off  InitialCurrent=0  Capacitance=470e-6  Setx0=on  InitialVoltage=0.1  Measurements=None
  Series RLC Branch3 : spsSeriesRLCBranchLib/Series RLC Branch  LConnTagsString=__new0  RConnTagsString=__new0  BranchType=C  Resistance=1  Inductance=1e-3  SetiL0=off  InitialCurrent=0  Capacitance=22e-6  Setx0=off  InitialVoltage=0  Measurements=None
  Series RLC Branch4 : spsSeriesRLCBranchLib/Series RLC Branch  LConnTagsString=__new0  RConnTagsString=__new0  BranchType=C  Resistance=1  Inductance=1e-3  SetiL0=off  InitialCurrent=0  Capacitance=470e-6  Setx0=on  InitialVoltage=0.1  Measurements=None
  V_out : Display
  V_pv : Display
  Voltage Measurement{,1..3} (4 alike) : spsVoltageMeasurementLib/Voltage Measurement  PhasorSimulation=off  OutputType=Complex  PSBequivalent=0
  Zero-Order Hold : ZeroOrderHold  SampleTime=0.05
  Zero-Order Hold1 : ZeroOrderHold  SampleTime=0.05
  Zero-Order Hold2 : ZeroOrderHold  SampleTime=0.05
  Ipv : Outport
  Vpv : Outport  Port=2
  Ppv : Outport  Port=3
  Iout : Outport  Port=4
  Vout : Outport  Port=5
  Pout : Outport  Port=6
  m : Outport  Port=7
  m1 : Outport  Port=8
  wires:
  Mean1/1 -> Ipv/1, I_pv/1
  Mean2/1 -> Vpv/1, V_pv/1
  PWM Generator (DC-DC)/1 -> Scope1/1, Mosfet/1
  Divide/1 -> Gain/1
  Current Measurement1/1 -> Product1/1, Mean5/1
  Constant1/1 -> MATLAB Function/2(T), PV Array/2
  Constant/1 -> MATLAB Function/1(G), PV Array/1
  Divide1/1 -> Gain1/1
  Gain1/1 -> Mean/1
  Voltage Measurement2/1 -> Scope/1
  Voltage Measurement/1 -> Product1/2, Mean7/1, Zero-Order Hold2/1
  Diode1/1 -> m/1
  Gain/1 -> Efisiensi Sistem/1
  P&O/1(D) -> Scope4/1, PWM Generator (DC-DC)/1
  Product/1 -> Mean3/1, Divide1/1
  Voltage Measurement1/1 -> Zero-Order Hold/1, Mean2/1, Product/2
  Current Measurement/1 -> Zero-Order Hold1/1, Product/1, Mean1/1
  Mean6/1 -> Divide/1, Pout/1, P_out/1
  Mean4/1 -> P_pv (calculation)/1
  Zero-Order Hold2/1 -> P&O/3(V_batt)
  Product1/1 -> Mean6/1
  Zero-Order Hold1/1 -> P&O/2(I_pv)
  Mean3/1 -> Ppv/1, P_pv (simulationl)/1, Divide/2
  Zero-Order Hold/1 -> P&O/1(V_pv)
  Mean5/1 -> Iout/1, I_out/1
  Voltage Measurement3/1 -> Scope3/1
  Mean7/1 -> Vout/1, V_out/1
  MATLAB Function/1(P_max) -> Mean4/1, Divide1/2
  Battery/1 -> Display2/1
  PV Array/1 -> Display1/1
  Mean/1 -> Efisiensi Daya (in)/1
  Mosfet/1 -> m1/1
  connections:
  Series RLC Branch3/RConn1 -- Diode1/LConn1 -- Series RLC Branch1/LConn1
  Series RLC Branch1/RConn1 -- Series RLC Branch4/RConn1 -- Voltage Measurement3/LConn2 -- PV Array/RConn2 -- Voltage Measurement1/LConn2 -- Mosfet/RConn1 -- Voltage Measurement2/LConn2 -- Voltage Measurement/LConn2 -- Battery/LConn2 -- Series RLC Branch2/RConn1
  PV Array/RConn1 -- Voltage Measurement3/LConn1 -- Voltage Measurement1/LConn1 -- Series RLC Branch4/LConn1 -- Current Measurement/LConn1
  Series RLC Branch/RConn1 -- Series RLC Branch3/LConn1 -- Mosfet/LConn1
  Current Measurement1/LConn1 -- Voltage Measurement2/LConn1 -- Series RLC Branch2/LConn1 -- Diode1/RConn1
  Current Measurement/RConn1 -- Series RLC Branch/LConn1
  Current Measurement1/RConn1 -- Voltage Measurement/LConn1 -- Battery/LConn1

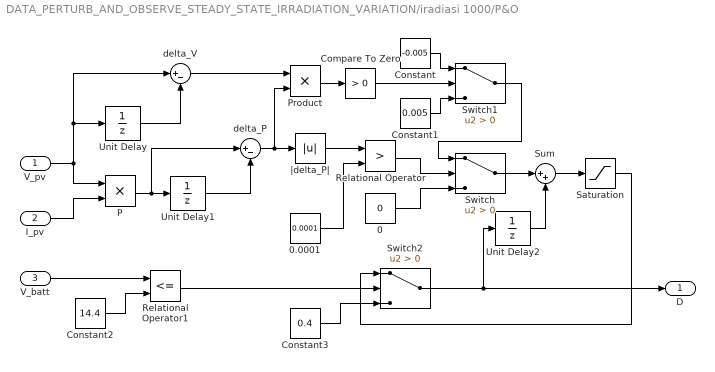
== system DATA_PERTURB_AND_OBSERVE_STEADY_STATE_IRRADIATION_VARIATION/iradiasi 1000/P&O ==
  V_pv : Inport
  I_pv : Inport  Port=2
  V_batt : Inport  Port=3
  0 : Constant  Value=0
  0.0001 : Constant  Value=0.0001
  Compare To Zero : simulink/Logic and Bit Operations/Compare To Zero  relop=>  OutDataTypeStr=boolean
  Constant : Constant  Value=-0.005
  Constant1 : Constant  Value=0.005
  Constant2 : Constant  Value=14.4
  Constant3 : Constant  Value=0.4
  P : Product
  Product : Product
  Relational Operator : RelationalOperator  Operator=>  OutDataTypeStr=boolean  RndMeth=Simplest  InputSameDT=off
  Relational Operator1 : RelationalOperator  Operator=<=  OutDataTypeStr=boolean  RndMeth=Simplest  InputSameDT=off
  Saturation : Saturate  UpperLimit=0.85  LowerLimit=0.15
  Sum : Sum  Inputs=|++
  Switch : Switch  Criteria=u2 > Threshold  SaturateOnIntegerOverflow=off  InputSameDT=off
  Switch1 : Switch  Criteria=u2 > Threshold  SaturateOnIntegerOverflow=off  InputSameDT=off
  Switch2 : Switch  Criteria=u2 > Threshold  SaturateOnIntegerOverflow=off  InputSameDT=off
  Unit Delay : UnitDelay  InitialCondition=21  SampleTime=-1  HasFrameUpgradeWarning=on
  Unit Delay1 : UnitDelay  SampleTime=-1  HasFrameUpgradeWarning=on
  Unit Delay2 : UnitDelay  InitialCondition=0.42  SampleTime=-1  HasFrameUpgradeWarning=on
  delta_P : Sum  Inputs=|+-
  delta_V : Sum  Inputs=|+-
  |delta_P| : Abs  SaturateOnIntegerOverflow=off
  D : Outport
  wires:
  Product/1 -> Compare To Zero/1
  Switch1/1 -> Switch/1
  Relational Operator1/1 -> Switch2/2
  Switch/1 -> Sum/1
  Switch2/1 -> D/1, Unit Delay2/1
  Constant2/1 -> Relational Operator1/2
  Saturation/1 -> Switch2/1
  Sum/1 -> Saturation/1
  delta_P/1 -> Product/2, |delta_P|/1
  Unit Delay2/1 -> Sum/2
  V_pv/1 -> P/1, delta_V/1, Unit Delay/1
  Constant1/1 -> Switch1/3
  delta_V/1 -> Product/1
  V_batt/1 -> Relational Operator1/1
  |delta_P|/1 -> Relational Operator/1
  0/1 -> Switch/3
  Unit Delay/1 -> delta_V/2
  I_pv/1 -> P/2
  Constant/1 -> Switch1/1
  Relational Operator/1 -> Switch/2
  Compare To Zero/1 -> Switch1/2
  P/1 -> delta_P/1, Unit Delay1/1
  0.0001/1 -> Relational Operator/2
  Constant3/1 -> Switch2/3
  Unit Delay1/1 -> delta_P/2

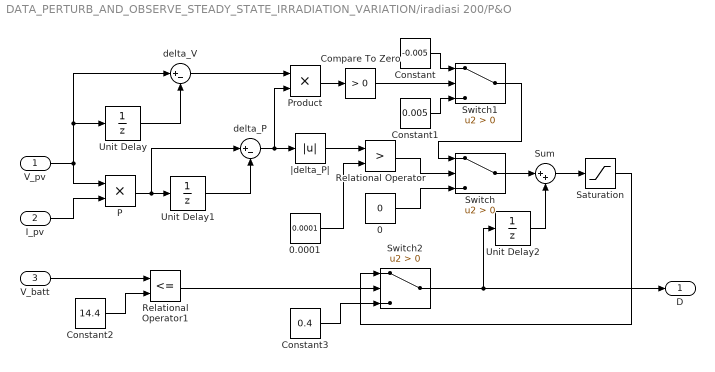
== system DATA_PERTURB_AND_OBSERVE_STEADY_STATE_IRRADIATION_VARIATION/iradiasi 200/P&O ==
  V_pv : Inport
  I_pv : Inport  Port=2
  V_batt : Inport  Port=3
  0 : Constant  Value=0
  0.0001 : Constant  Value=0.0001
  Compare To Zero : simulink/Logic and Bit Operations/Compare To Zero  relop=>  OutDataTypeStr=boolean
  Constant : Constant  Value=-0.005
  Constant1 : Constant  Value=0.005
  Constant2 : Constant  Value=14.4
  Constant3 : Constant  Value=0.4
  P : Product
  Product : Product
  Relational Operator : RelationalOperator  Operator=>  OutDataTypeStr=boolean  RndMeth=Simplest  InputSameDT=off
  Relational Operator1 : RelationalOperator  Operator=<=  OutDataTypeStr=boolean  RndMeth=Simplest  InputSameDT=off
  Saturation : Saturate  UpperLimit=0.85  LowerLimit=0.15
  Sum : Sum  Inputs=|++
  Switch : Switch  Criteria=u2 > Threshold  SaturateOnIntegerOverflow=off  InputSameDT=off
  Switch1 : Switch  Criteria=u2 > Threshold  SaturateOnIntegerOverflow=off  InputSameDT=off
  Switch2 : Switch  Criteria=u2 > Threshold  SaturateOnIntegerOverflow=off  InputSameDT=off
  Unit Delay : UnitDelay  InitialCondition=21  SampleTime=-1  HasFrameUpgradeWarning=on
  Unit Delay1 : UnitDelay  SampleTime=-1  HasFrameUpgradeWarning=on
  Unit Delay2 : UnitDelay  InitialCondition=0.42  SampleTime=-1  HasFrameUpgradeWarning=on
  delta_P : Sum  Inputs=|+-
  delta_V : Sum  Inputs=|+-
  |delta_P| : Abs  SaturateOnIntegerOverflow=off
  D : Outport
  wires:
  Product/1 -> Compare To Zero/1
  Switch1/1 -> Switch/1
  Relational Operator1/1 -> Switch2/2
  Switch/1 -> Sum/1
  Switch2/1 -> D/1, Unit Delay2/1
  Constant2/1 -> Relational Operator1/2
  Saturation/1 -> Switch2/1
  Sum/1 -> Saturation/1
  delta_P/1 -> Product/2, |delta_P|/1
  Unit Delay2/1 -> Sum/2
  V_pv/1 -> P/1, delta_V/1, Unit Delay/1
  Constant1/1 -> Switch1/3
  delta_V/1 -> Product/1
  V_batt/1 -> Relational Operator1/1
  |delta_P|/1 -> Relational Operator/1
  0/1 -> Switch/3
  Unit Delay/1 -> delta_V/2
  I_pv/1 -> P/2
  Constant/1 -> Switch1/1
  Relational Operator/1 -> Switch/2
  Compare To Zero/1 -> Switch1/2
  P/1 -> delta_P/1, Unit Delay1/1
  0.0001/1 -> Relational Operator/2
  Constant3/1 -> Switch2/3
  Unit Delay1/1 -> delta_P/2

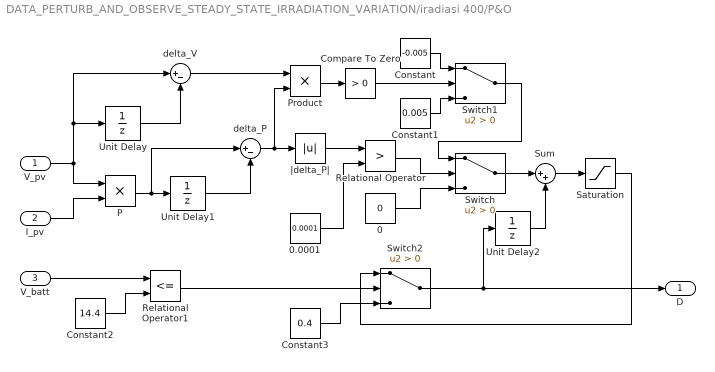
== system DATA_PERTURB_AND_OBSERVE_STEADY_STATE_IRRADIATION_VARIATION/iradiasi 400/P&O ==
  V_pv : Inport
  I_pv : Inport  Port=2
  V_batt : Inport  Port=3
  0 : Constant  Value=0
  0.0001 : Constant  Value=0.0001
  Compare To Zero : simulink/Logic and Bit Operations/Compare To Zero  relop=>  OutDataTypeStr=boolean
  Constant : Constant  Value=-0.005
  Constant1 : Constant  Value=0.005
  Constant2 : Constant  Value=14.4
  Constant3 : Constant  Value=0.4
  P : Product
  Product : Product
  Relational Operator : RelationalOperator  Operator=>  OutDataTypeStr=boolean  RndMeth=Simplest  InputSameDT=off
  Relational Operator1 : RelationalOperator  Operator=<=  OutDataTypeStr=boolean  RndMeth=Simplest  InputSameDT=off
  Saturation : Saturate  UpperLimit=0.85  LowerLimit=0.15
  Sum : Sum  Inputs=|++
  Switch : Switch  Criteria=u2 > Threshold  SaturateOnIntegerOverflow=off  InputSameDT=off
  Switch1 : Switch  Criteria=u2 > Threshold  SaturateOnIntegerOverflow=off  InputSameDT=off
  Switch2 : Switch  Criteria=u2 > Threshold  SaturateOnIntegerOverflow=off  InputSameDT=off
  Unit Delay : UnitDelay  InitialCondition=21  SampleTime=-1  HasFrameUpgradeWarning=on
  Unit Delay1 : UnitDelay  SampleTime=-1  HasFrameUpgradeWarning=on
  Unit Delay2 : UnitDelay  InitialCondition=0.42  SampleTime=-1  HasFrameUpgradeWarning=on
  delta_P : Sum  Inputs=|+-
  delta_V : Sum  Inputs=|+-
  |delta_P| : Abs  SaturateOnIntegerOverflow=off
  D : Outport
  wires:
  Product/1 -> Compare To Zero/1
  Switch1/1 -> Switch/1
  Relational Operator1/1 -> Switch2/2
  Switch/1 -> Sum/1
  Switch2/1 -> D/1, Unit Delay2/1
  Constant2/1 -> Relational Operator1/2
  Saturation/1 -> Switch2/1
  Sum/1 -> Saturation/1
  delta_P/1 -> Product/2, |delta_P|/1
  Unit Delay2/1 -> Sum/2
  V_pv/1 -> P/1, delta_V/1, Unit Delay/1
  Constant1/1 -> Switch1/3
  delta_V/1 -> Product/1
  V_batt/1 -> Relational Operator1/1
  |delta_P|/1 -> Relational Operator/1
  0/1 -> Switch/3
  Unit Delay/1 -> delta_V/2
  I_pv/1 -> P/2
  Constant/1 -> Switch1/1
  Relational Operator/1 -> Switch/2
  Compare To Zero/1 -> Switch1/2
  P/1 -> delta_P/1, Unit Delay1/1
  0.0001/1 -> Relational Operator/2
  Constant3/1 -> Switch2/3
  Unit Delay1/1 -> delta_P/2

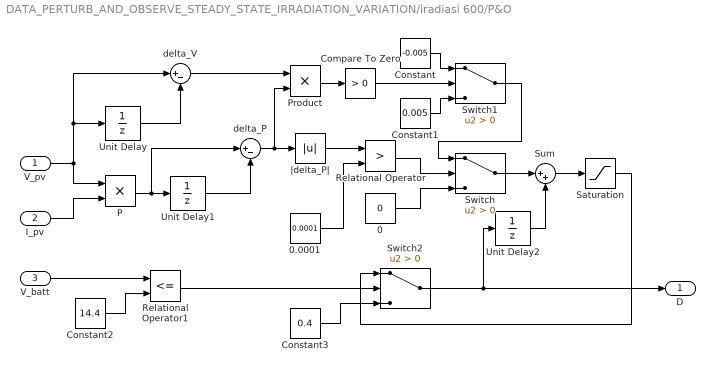
== system DATA_PERTURB_AND_OBSERVE_STEADY_STATE_IRRADIATION_VARIATION/iradiasi 600/P&O ==
  V_pv : Inport
  I_pv : Inport  Port=2
  V_batt : Inport  Port=3
  0 : Constant  Value=0
  0.0001 : Constant  Value=0.0001
  Compare To Zero : simulink/Logic and Bit Operations/Compare To Zero  relop=>  OutDataTypeStr=boolean
  Constant : Constant  Value=-0.005
  Constant1 : Constant  Value=0.005
  Constant2 : Constant  Value=14.4
  Constant3 : Constant  Value=0.4
  P : Product
  Product : Product
  Relational Operator : RelationalOperator  Operator=>  OutDataTypeStr=boolean  RndMeth=Simplest  InputSameDT=off
  Relational Operator1 : RelationalOperator  Operator=<=  OutDataTypeStr=boolean  RndMeth=Simplest  InputSameDT=off
  Saturation : Saturate  UpperLimit=0.85  LowerLimit=0.15
  Sum : Sum  Inputs=|++
  Switch : Switch  Criteria=u2 > Threshold  SaturateOnIntegerOverflow=off  InputSameDT=off
  Switch1 : Switch  Criteria=u2 > Threshold  SaturateOnIntegerOverflow=off  InputSameDT=off
  Switch2 : Switch  Criteria=u2 > Threshold  SaturateOnIntegerOverflow=off  InputSameDT=off
  Unit Delay : UnitDelay  InitialCondition=21  SampleTime=-1  HasFrameUpgradeWarning=on
  Unit Delay1 : UnitDelay  SampleTime=-1  HasFrameUpgradeWarning=on
  Unit Delay2 : UnitDelay  InitialCondition=0.42  SampleTime=-1  HasFrameUpgradeWarning=on
  delta_P : Sum  Inputs=|+-
  delta_V : Sum  Inputs=|+-
  |delta_P| : Abs  SaturateOnIntegerOverflow=off
  D : Outport
  wires:
  Product/1 -> Compare To Zero/1
  Switch1/1 -> Switch/1
  Relational Operator1/1 -> Switch2/2
  Switch/1 -> Sum/1
  Switch2/1 -> D/1, Unit Delay2/1
  Constant2/1 -> Relational Operator1/2
  Saturation/1 -> Switch2/1
  Sum/1 -> Saturation/1
  delta_P/1 -> Product/2, |delta_P|/1
  Unit Delay2/1 -> Sum/2
  V_pv/1 -> P/1, delta_V/1, Unit Delay/1
  Constant1/1 -> Switch1/3
  delta_V/1 -> Product/1
  V_batt/1 -> Relational Operator1/1
  |delta_P|/1 -> Relational Operator/1
  0/1 -> Switch/3
  Unit Delay/1 -> delta_V/2
  I_pv/1 -> P/2
  Constant/1 -> Switch1/1
  Relational Operator/1 -> Switch/2
  Compare To Zero/1 -> Switch1/2
  P/1 -> delta_P/1, Unit Delay1/1
  0.0001/1 -> Relational Operator/2
  Constant3/1 -> Switch2/3
  Unit Delay1/1 -> delta_P/2

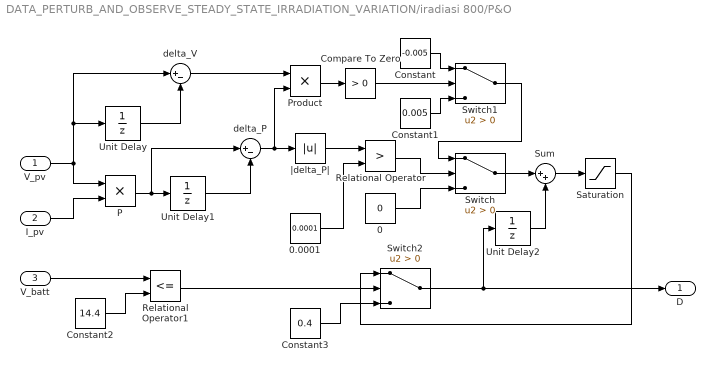
== system DATA_PERTURB_AND_OBSERVE_STEADY_STATE_IRRADIATION_VARIATION/iradiasi 800/P&O ==
  V_pv : Inport
  I_pv : Inport  Port=2
  V_batt : Inport  Port=3
  0 : Constant  Value=0
  0.0001 : Constant  Value=0.0001
  Compare To Zero : simulink/Logic and Bit Operations/Compare To Zero  relop=>  OutDataTypeStr=boolean
  Constant : Constant  Value=-0.005
  Constant1 : Constant  Value=0.005
  Constant2 : Constant  Value=14.4
  Constant3 : Constant  Value=0.4
  P : Product
  Product : Product
  Relational Operator : RelationalOperator  Operator=>  OutDataTypeStr=boolean  RndMeth=Simplest  InputSameDT=off
  Relational Operator1 : RelationalOperator  Operator=<=  OutDataTypeStr=boolean  RndMeth=Simplest  InputSameDT=off
  Saturation : Saturate  UpperLimit=0.85  LowerLimit=0.15
  Sum : Sum  Inputs=|++
  Switch : Switch  Criteria=u2 > Threshold  SaturateOnIntegerOverflow=off  InputSameDT=off
  Switch1 : Switch  Criteria=u2 > Threshold  SaturateOnIntegerOverflow=off  InputSameDT=off
  Switch2 : Switch  Criteria=u2 > Threshold  SaturateOnIntegerOverflow=off  InputSameDT=off
  Unit Delay : UnitDelay  InitialCondition=21  SampleTime=-1  HasFrameUpgradeWarning=on
  Unit Delay1 : UnitDelay  SampleTime=-1  HasFrameUpgradeWarning=on
  Unit Delay2 : UnitDelay  InitialCondition=0.42  SampleTime=-1  HasFrameUpgradeWarning=on
  delta_P : Sum  Inputs=|+-
  delta_V : Sum  Inputs=|+-
  |delta_P| : Abs  SaturateOnIntegerOverflow=off
  D : Outport
  wires:
  Product/1 -> Compare To Zero/1
  Switch1/1 -> Switch/1
  Relational Operator1/1 -> Switch2/2
  Switch/1 -> Sum/1
  Switch2/1 -> D/1, Unit Delay2/1
  Constant2/1 -> Relational Operator1/2
  Saturation/1 -> Switch2/1
  Sum/1 -> Saturation/1
  delta_P/1 -> Product/2, |delta_P|/1
  Unit Delay2/1 -> Sum/2
  V_pv/1 -> P/1, delta_V/1, Unit Delay/1
  Constant1/1 -> Switch1/3
  delta_V/1 -> Product/1
  V_batt/1 -> Relational Operator1/1
  |delta_P|/1 -> Relational Operator/1
  0/1 -> Switch/3
  Unit Delay/1 -> delta_V/2
  I_pv/1 -> P/2
  Constant/1 -> Switch1/1
  Relational Operator/1 -> Switch/2
  Compare To Zero/1 -> Switch1/2
  P/1 -> delta_P/1, Unit Delay1/1
  0.0001/1 -> Relational Operator/2
  Constant3/1 -> Switch2/3
  Unit Delay1/1 -> delta_P/2

== matlab function DATA_PERTURB_AND_OBSERVE_STEADY_STATE_IRRADIATION_VARIATION/iradiasi 1000/MATLAB Function ==
  data: G input; P_max output; T input
function P_max = Pmax_Teori(G, T)
    % Parameter PV Array Piksel Liar / User-Defined
    P_stc = 10.08;   % Daya Maksimum (Watt)
    G_stc = 1000;    % Iradiasi standar (W/m^2)
    T_stc = 25;      % Suhu standar (Celcius)
    
    % Koefisien suhu untuk daya (dalam desimal)
    gamma = -0.0025899; 
    
    % Perhitungan Daya Maksimum Teoritis Dinamis
    P_max = P_stc * (G/G_stc) * (1 + gamma * (T - T_stc));
end

== matlab function DATA_PERTURB_AND_OBSERVE_STEADY_STATE_IRRADIATION_VARIATION/iradiasi 600/MATLAB Function ==
  data: G input; P_max output; T input
function P_max = Pmax_Teori(G, T)
    % Parameter PV Array Piksel Liar / User-Defined
    P_stc = 10.08;   % Daya Maksimum (Watt)
    G_stc = 1000;    % Iradiasi standar (W/m^2)
    T_stc = 25;      % Suhu standar (Celcius)
    
    % Koefisien suhu untuk daya (dalam desimal)
    gamma = -0.0025899; 
    
    % Perhitungan Daya Maksimum Teoritis Dinamis
    P_max = P_stc * (G/G_stc) * (1 + gamma * (T - T_stc));
end

== matlab function DATA_PERTURB_AND_OBSERVE_STEADY_STATE_IRRADIATION_VARIATION/iradiasi 400/MATLAB Function ==
  data: G input; P_max output; T input
function P_max = Pmax_Teori(G, T)
    % Parameter PV Array Piksel Liar / User-Defined
    P_stc = 10.08;   % Daya Maksimum (Watt)
    G_stc = 1000;    % Iradiasi standar (W/m^2)
    T_stc = 25;      % Suhu standar (Celcius)
    
    % Koefisien suhu untuk daya (dalam desimal)
    gamma = -0.0025899; 
    
    % Perhitungan Daya Maksimum Teoritis Dinamis
    P_max = P_stc * (G/G_stc) * (1 + gamma * (T - T_stc));
end

== matlab function DATA_PERTURB_AND_OBSERVE_STEADY_STATE_IRRADIATION_VARIATION/iradiasi 200/MATLAB Function ==
  data: G input; P_max output; T input
function P_max = Pmax_Teori(G, T)
    % Parameter PV Array Piksel Liar / User-Defined
    P_stc = 10.08;   % Daya Maksimum (Watt)
    G_stc = 1000;    % Iradiasi standar (W/m^2)
    T_stc = 25;      % Suhu standar (Celcius)
    
    % Koefisien suhu untuk daya (dalam desimal)
    gamma = -0.0025899; 
    
    % Perhitungan Daya Maksimum Teoritis Dinamis
    P_max = P_stc * (G/G_stc) * (1 + gamma * (T - T_stc));
end

== matlab function DATA_PERTURB_AND_OBSERVE_STEADY_STATE_IRRADIATION_VARIATION/iradiasi 800/MATLAB Function ==
  data: G input; P_max output; T input
function P_max = Pmax_Teori(G, T)
    % Parameter PV Array Piksel Liar / User-Defined
    P_stc = 10.08;   % Daya Maksimum (Watt)
    G_stc = 1000;    % Iradiasi standar (W/m^2)
    T_stc = 25;      % Suhu standar (Celcius)
    
    % Koefisien suhu untuk daya (dalam desimal)
    gamma = -0.0025899; 
    
    % Perhitungan Daya Maksimum Teoritis Dinamis
    P_max = P_stc * (G/G_stc) * (1 + gamma * (T - T_stc));
end
